simulink model "chaine_qpsk_hamming"  (R2023b)
settings: Solver=FixedStepDiscrete  StartTime=0.0  StopTime=(N/8 - 1)*8*Tb  FixedStep=8*Tb  RelTol=1e-3
values from neighbouring files (symbols this model uses):
  graine = P.graine    [parametres.m]    (also in parametres_perso.m = mod(sum(c .* (1:numel(c)) * 31) + 7 * numel(c), 2^31 - 1); partie2_1.m)
  N0 = Es / (2*g)    (= 0.158113883008)    [creer_qpsk.m]    (also in creer_qpsk_hamming.m = 0.276699295265; parametres.m = Eb / 10^(EbN0dB/10))
  Tb = 1    [parametres.m]    (also in partie2_1.m)
libraries: simulink x3
settings Model: Creator=e2507477  LastModifiedBy=e2507477

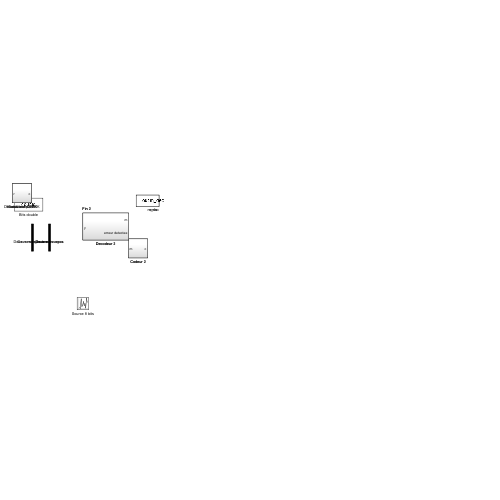
[thumbnail: Simulink's stored preview of the top-level diagram]
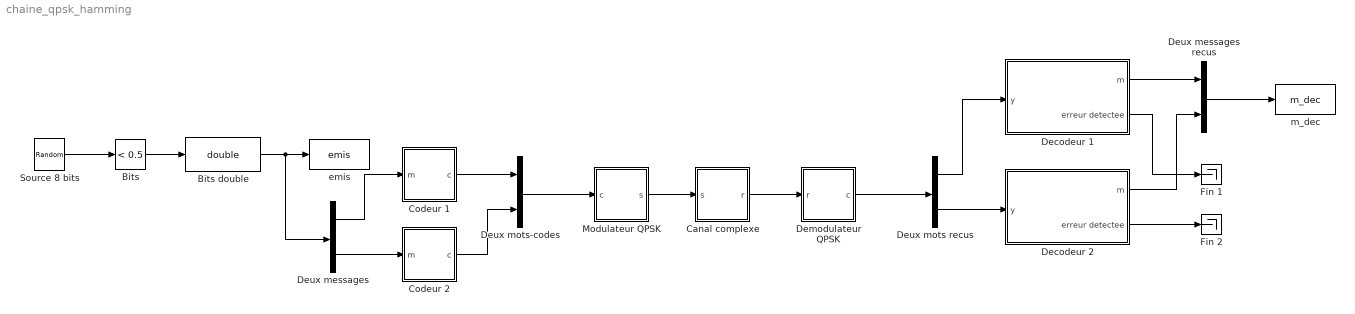
== system chaine_qpsk_hamming ==
  Bits : simulink/Logic and Bit Operations/Compare To Constant  relop=<  const=0.5  OutDataTypeStr=boolean
  Bits double : DataTypeConversion  OutDataTypeStr=double  SaturateOnIntegerOverflow=off  RndMeth=Floor
  Canal complexe : Subsystem
  Codeur 1 : Subsystem
  Codeur 2 : Subsystem
  Decodeur 1 : Subsystem
  Decodeur 2 : Subsystem
  Demodulateur QPSK : Subsystem
  Deux messages : Demux  Outputs=[4 4]
  Deux messages recus : Mux  Inputs=2
  Deux mots recus : Demux  Outputs=[7 7]
  Deux mots-codes : Mux  Inputs=2
  Fin 1 : Terminator
  Fin 2 : Terminator
  Modulateur QPSK : Subsystem
  Source 8 bits : UniformRandomNumber  Minimum=zeros(1,8)  Maximum=ones(1,8)  Seed=round(graine) + 7919*(0:7)  SampleTime=8*Tb
  emis : ToWorkspace  VariableName=emis  SampleTime=-1
  m_dec : ToWorkspace  VariableName=m_dec  SampleTime=-1
  wires:
  Bits/1 -> Bits double/1
  Source 8 bits/1 -> Bits/1
  Deux messages/2 -> Codeur 2/1(m)
  Deux messages/1 -> Codeur 1/1(m)
  Bits double/1 -> Deux messages/1, emis/1
  Demodulateur QPSK/1(c) -> Deux mots recus/1
  Codeur 1/1(c) -> Deux mots-codes/1
  Deux mots-codes/1 -> Modulateur QPSK/1(c)
  Codeur 2/1(c) -> Deux mots-codes/2
  Modulateur QPSK/1(s) -> Canal complexe/1(s)
  Canal complexe/1(r) -> Demodulateur QPSK/1(r)
  Deux mots recus/1 -> Decodeur 1/1(y)
  Deux mots recus/2 -> Decodeur 2/1(y)
  Decodeur 1/1(m) -> Deux messages recus/1
  Decodeur 1/2(erreur detectee) -> Fin 1/1
  Decodeur 2/1(m) -> Deux messages recus/2
  Decodeur 2/2(erreur detectee) -> Fin 2/1
  Deux messages recus/1 -> m_dec/1

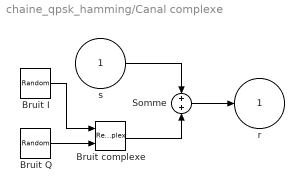
== system chaine_qpsk_hamming/Canal complexe ==
  s : Inport
  Bruit I : RandomNumber  Mean=zeros(1,7)  Variance=N0/2*ones(1,7)  Seed=round(graine) + 50000 + 7919*(0:6)  SampleTime=8*Tb
  Bruit Q : RandomNumber  Mean=zeros(1,7)  Variance=N0/2*ones(1,7)  Seed=round(graine) + 90000 + 7919*(0:6)  SampleTime=8*Tb
  Bruit complexe : RealImagToComplex
  Somme : Sum
  r : Outport
  wires:
  Somme/1 -> r/1
  Bruit complexe/1 -> Somme/2
  s/1 -> Somme/1
  Bruit Q/1 -> Bruit complexe/2
  Bruit I/1 -> Bruit complexe/1

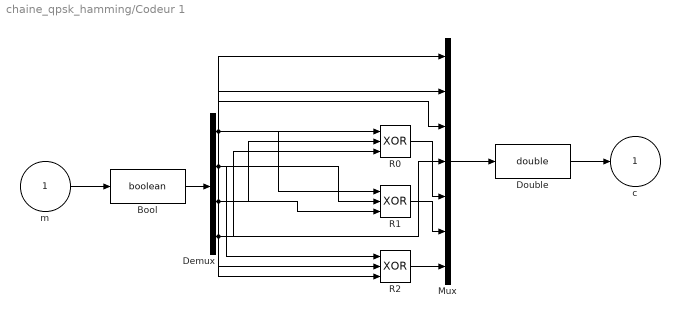
== system chaine_qpsk_hamming/Codeur 1 ==
  m : Inport
  Bool : DataTypeConversion  OutDataTypeStr=boolean  SaturateOnIntegerOverflow=off  RndMeth=Floor
  Demux : Demux
  Double : DataTypeConversion  OutDataTypeStr=double  SaturateOnIntegerOverflow=off  RndMeth=Floor
  Mux : Mux  Inputs=7
  R0 : Logic  Operator=XOR  Inputs=3  AllPortsSameDT=off  OutDataTypeStr=boolean
  R1 : Logic  Operator=XOR  Inputs=3  AllPortsSameDT=off  OutDataTypeStr=boolean
  R2 : Logic  Operator=XOR  Inputs=3  AllPortsSameDT=off  OutDataTypeStr=boolean
  c : Outport
  wires:
  Mux/1 -> Double/1
  Double/1 -> c/1
  R2/1 -> Mux/7
  R0/1 -> Mux/5
  R1/1 -> Mux/6
  Demux/3 -> R2/2, R1/3, R0/2, Mux/3
  Demux/4 -> Mux/4, R2/3, R0/3
  Bool/1 -> Demux/1
  Demux/1 -> R1/1, R0/1, Mux/1
  Demux/2 -> R2/1, R1/2, Mux/2
  m/1 -> Bool/1

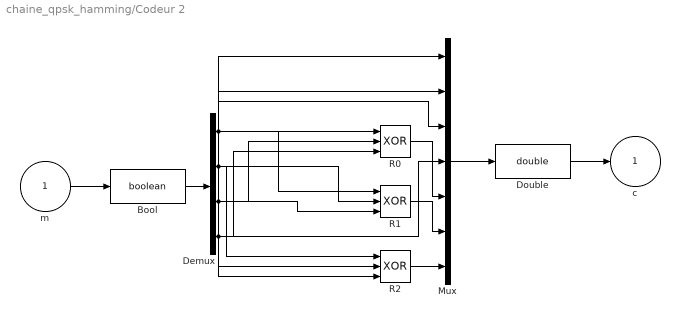
== system chaine_qpsk_hamming/Codeur 2 ==
  m : Inport
  Bool : DataTypeConversion  OutDataTypeStr=boolean  SaturateOnIntegerOverflow=off  RndMeth=Floor
  Demux : Demux
  Double : DataTypeConversion  OutDataTypeStr=double  SaturateOnIntegerOverflow=off  RndMeth=Floor
  Mux : Mux  Inputs=7
  R0 : Logic  Operator=XOR  Inputs=3  AllPortsSameDT=off  OutDataTypeStr=boolean
  R1 : Logic  Operator=XOR  Inputs=3  AllPortsSameDT=off  OutDataTypeStr=boolean
  R2 : Logic  Operator=XOR  Inputs=3  AllPortsSameDT=off  OutDataTypeStr=boolean
  c : Outport
  wires:
  Mux/1 -> Double/1
  Double/1 -> c/1
  R2/1 -> Mux/7
  R0/1 -> Mux/5
  R1/1 -> Mux/6
  Demux/3 -> R2/2, R1/3, R0/2, Mux/3
  Demux/4 -> Mux/4, R2/3, R0/3
  Bool/1 -> Demux/1
  Demux/1 -> R1/1, R0/1, Mux/1
  Demux/2 -> R2/1, R1/2, Mux/2
  m/1 -> Bool/1

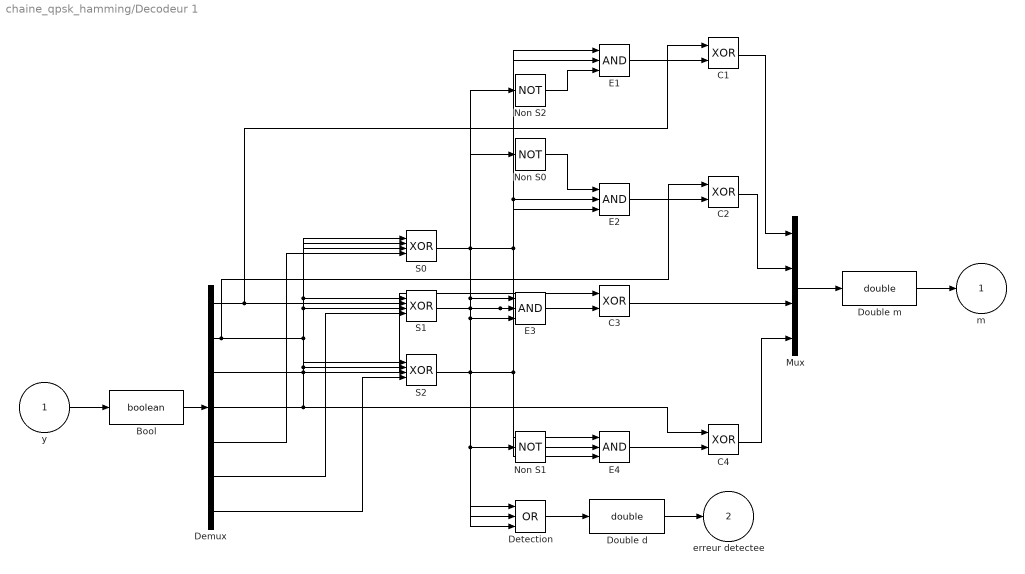
== system chaine_qpsk_hamming/Decodeur 1 ==
  y : Inport
  Bool : DataTypeConversion  OutDataTypeStr=boolean  SaturateOnIntegerOverflow=off  RndMeth=Floor
  C{1..4} (4 alike) : Logic  Operator=XOR  AllPortsSameDT=off  OutDataTypeStr=boolean
  Demux : Demux  Outputs=7
  Detection : Logic  Operator=OR  Inputs=3  AllPortsSameDT=off  OutDataTypeStr=boolean
  Double d : DataTypeConversion  OutDataTypeStr=double  SaturateOnIntegerOverflow=off  RndMeth=Floor
  Double m : DataTypeConversion  OutDataTypeStr=double  SaturateOnIntegerOverflow=off  RndMeth=Floor
  E{1..4} (4 alike) : Logic  Inputs=3  AllPortsSameDT=off  OutDataTypeStr=boolean
  Mux : Mux
  Non S0 : Logic  Operator=NOT  AllPortsSameDT=off  OutDataTypeStr=boolean
  Non S1 : Logic  Operator=NOT  AllPortsSameDT=off  OutDataTypeStr=boolean
  Non S2 : Logic  Operator=NOT  AllPortsSameDT=off  OutDataTypeStr=boolean
  S0 : Logic  Operator=XOR  Inputs=4  AllPortsSameDT=off  OutDataTypeStr=boolean
  S1 : Logic  Operator=XOR  Inputs=4  AllPortsSameDT=off  OutDataTypeStr=boolean
  S2 : Logic  Operator=XOR  Inputs=4  AllPortsSameDT=off  OutDataTypeStr=boolean
  m : Outport
  erreur detectee : Outport  Port=2
  wires:
  Double m/1 -> m/1
  Mux/1 -> Double m/1
  C4/1 -> Mux/4
  C2/1 -> Mux/2
  C1/1 -> Mux/1
  Double d/1 -> erreur detectee/1
  E4/1 -> C4/2
  C3/1 -> Mux/3
  E2/1 -> C2/2
  E1/1 -> C1/2
  E3/1 -> C3/2
  Non S2/1 -> E1/3
  S2/1 -> Detection/3, Non S2/1, E3/3, E4/3, E2/3
  Demux/7 -> S2/4
  S0/1 -> Non S0/1, E4/1, E1/1, E3/1, Detection/1
  S1/1 -> E3/2, E2/2, E1/2, Detection/2, Non S1/1
  Demux/5 -> S0/4
  Detection/1 -> Double d/1
  Demux/1 -> C1/1, S1/1, S0/1
  Demux/3 -> C3/1, S2/2, S1/3, S0/2
  Demux/6 -> S1/4
  y/1 -> Bool/1
  Bool/1 -> Demux/1
  Demux/2 -> C2/1, S1/2, S2/1
  Non S0/1 -> E2/1
  Non S1/1 -> E4/2
  Demux/4 -> C4/1, S2/3, S0/3

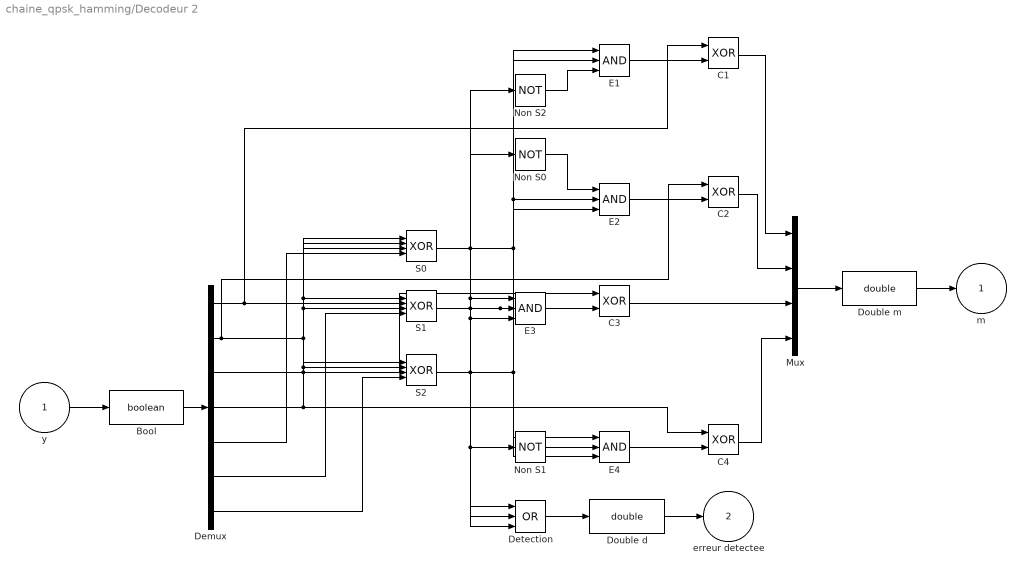
== system chaine_qpsk_hamming/Decodeur 2 ==
  y : Inport
  Bool : DataTypeConversion  OutDataTypeStr=boolean  SaturateOnIntegerOverflow=off  RndMeth=Floor
  C{1..4} (4 alike) : Logic  Operator=XOR  AllPortsSameDT=off  OutDataTypeStr=boolean
  Demux : Demux  Outputs=7
  Detection : Logic  Operator=OR  Inputs=3  AllPortsSameDT=off  OutDataTypeStr=boolean
  Double d : DataTypeConversion  OutDataTypeStr=double  SaturateOnIntegerOverflow=off  RndMeth=Floor
  Double m : DataTypeConversion  OutDataTypeStr=double  SaturateOnIntegerOverflow=off  RndMeth=Floor
  E{1..4} (4 alike) : Logic  Inputs=3  AllPortsSameDT=off  OutDataTypeStr=boolean
  Mux : Mux
  Non S0 : Logic  Operator=NOT  AllPortsSameDT=off  OutDataTypeStr=boolean
  Non S1 : Logic  Operator=NOT  AllPortsSameDT=off  OutDataTypeStr=boolean
  Non S2 : Logic  Operator=NOT  AllPortsSameDT=off  OutDataTypeStr=boolean
  S0 : Logic  Operator=XOR  Inputs=4  AllPortsSameDT=off  OutDataTypeStr=boolean
  S1 : Logic  Operator=XOR  Inputs=4  AllPortsSameDT=off  OutDataTypeStr=boolean
  S2 : Logic  Operator=XOR  Inputs=4  AllPortsSameDT=off  OutDataTypeStr=boolean
  m : Outport
  erreur detectee : Outport  Port=2
  wires:
  Double m/1 -> m/1
  Mux/1 -> Double m/1
  C4/1 -> Mux/4
  C2/1 -> Mux/2
  C1/1 -> Mux/1
  Double d/1 -> erreur detectee/1
  E4/1 -> C4/2
  C3/1 -> Mux/3
  E2/1 -> C2/2
  E1/1 -> C1/2
  E3/1 -> C3/2
  Non S2/1 -> E1/3
  S2/1 -> Detection/3, Non S2/1, E3/3, E4/3, E2/3
  Demux/7 -> S2/4
  S0/1 -> Non S0/1, E4/1, E1/1, E3/1, Detection/1
  S1/1 -> E3/2, E2/2, E1/2, Detection/2, Non S1/1
  Demux/5 -> S0/4
  Detection/1 -> Double d/1
  Demux/1 -> C1/1, S1/1, S0/1
  Demux/3 -> C3/1, S2/2, S1/3, S0/2
  Demux/6 -> S1/4
  y/1 -> Bool/1
  Bool/1 -> Demux/1
  Demux/2 -> C2/1, S1/2, S2/1
  Non S0/1 -> E2/1
  Non S1/1 -> E4/2
  Demux/4 -> C4/1, S2/3, S0/3

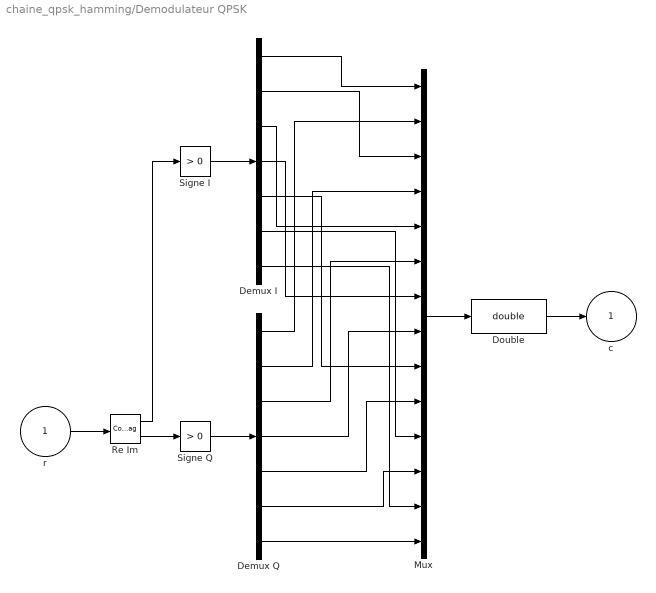
== system chaine_qpsk_hamming/Demodulateur QPSK ==
  r : Inport
  Demux I : Demux  Outputs=7
  Demux Q : Demux  Outputs=7
  Double : DataTypeConversion  OutDataTypeStr=double  SaturateOnIntegerOverflow=off  RndMeth=Floor
  Mux : Mux  Inputs=14
  Re Im : ComplexToRealImag
  Signe I : simulink/Logic and Bit Operations/Compare To Constant  relop=>  const=0  OutDataTypeStr=boolean
  Signe Q : simulink/Logic and Bit Operations/Compare To Constant  relop=>  const=0  OutDataTypeStr=boolean
  c : Outport
  wires:
  r/1 -> Re Im/1
  Re Im/1 -> Signe I/1
  Demux I/1 -> Mux/1
  Signe Q/1 -> Demux Q/1
  Signe I/1 -> Demux I/1
  Re Im/2 -> Signe Q/1
  Demux I/2 -> Mux/3
  Demux I/3 -> Mux/5
  Double/1 -> c/1
  Demux I/4 -> Mux/7
  Demux I/5 -> Mux/9
  Demux I/6 -> Mux/11
  Demux I/7 -> Mux/13
  Demux Q/1 -> Mux/2
  Demux Q/2 -> Mux/4
  Mux/1 -> Double/1
  Demux Q/3 -> Mux/6
  Demux Q/4 -> Mux/8
  Demux Q/5 -> Mux/10
  Demux Q/6 -> Mux/12
  Demux Q/7 -> Mux/14

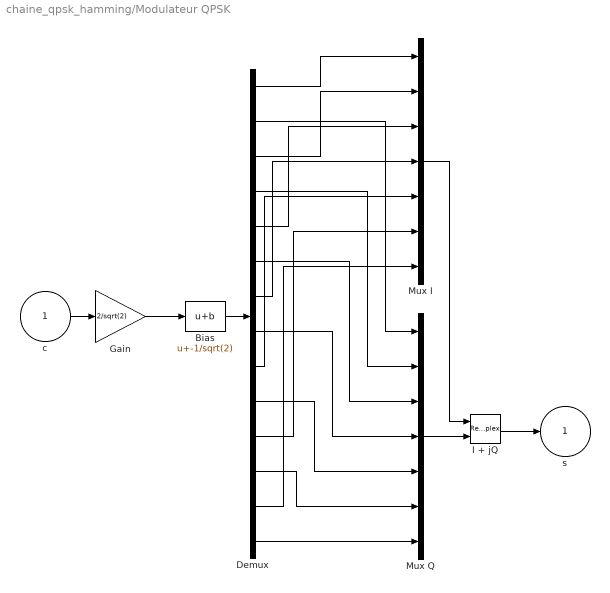
== system chaine_qpsk_hamming/Modulateur QPSK ==
  c : Inport
  Bias : Bias  Bias=-1/sqrt(2)  SaturateOnIntegerOverflow=off
  Demux : Demux  Outputs=14
  Gain : Gain  Gain=2/sqrt(2)
  I + jQ : RealImagToComplex
  Mux I : Mux  Inputs=7
  Mux Q : Mux  Inputs=7
  s : Outport
  wires:
  Demux/5 -> Mux I/3
  c/1 -> Gain/1
  Demux/4 -> Mux Q/2
  Demux/3 -> Mux I/2
  Gain/1 -> Bias/1
  Demux/2 -> Mux Q/1
  Demux/1 -> Mux I/1
  Demux/14 -> Mux Q/7
  Bias/1 -> Demux/1
  Demux/6 -> Mux Q/3
  Demux/7 -> Mux I/4
  Demux/8 -> Mux Q/4
  Demux/9 -> Mux I/5
  Demux/10 -> Mux Q/5
  Demux/11 -> Mux I/6
  Demux/12 -> Mux Q/6
  Demux/13 -> Mux I/7
  Mux I/1 -> I + jQ/1
  Mux Q/1 -> I + jQ/2
  I + jQ/1 -> s/1
